simulink model "fixed_point_model"  (R2022b)
settings: Solver=FixedStepDiscrete  StartTime=0.0  StopTime=0.01  FixedStep=1e-10  RelTol=1e-3
undefined symbols (not defined in the file or in its folder): theta_input
libraries: dspsigops x206, dspsrcs4 x16, simulink x8, commdigbbndpm3 x1, commrandsrc3 x1
(part 1 of 6)
settings Model: FPTShortcutValueString='{{},{''BaselineRun'',1,1,1,''BaselineRun'','''',{},''M'','''',''''}}'  Creator=ASAA  LastModifiedBy=ASAA
settings DataIOCC: SaveOutput=off  SignalLogging=off  DSMLogging=off  ReturnWorkspaceOutputs=off
settings DebuggingCC: SignalRangeChecking=warning  UnderSpecifiedDimensionMsg=warning

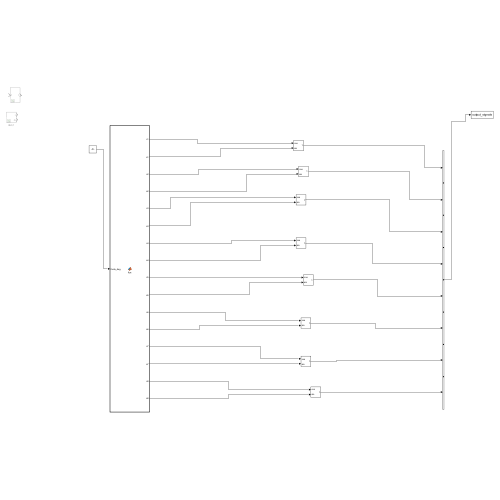
[thumbnail: Simulink's stored preview of the top-level diagram]
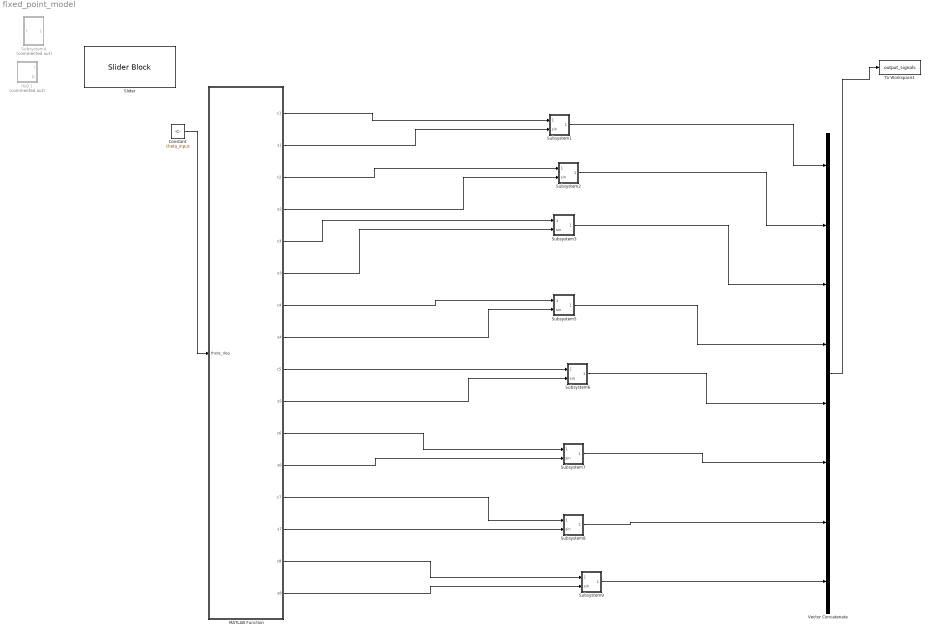
== system fixed_point_model ==
  Constant : Constant  Value=theta_input
  I&Q 1 : Subsystem  Commented=on
  MATLAB Function : MATLAB Function  TreatAsAtomicUnit=on
  Slider : SliderBlock
  Subsystem1 : Subsystem
  Subsystem2 : Subsystem
  Subsystem3 : Subsystem
  Subsystem4 : Subsystem  Commented=on
  Subsystem5 : Subsystem
  Subsystem6 : Subsystem
  Subsystem7 : Subsystem
  Subsystem8 : Subsystem
  Subsystem9 : Subsystem
  To Workspace1 : ToWorkspace  VariableName=output_signals  SampleTime=-1
  Vector Concatenate : Concatenate  NumInputs=8
  wires:
  Constant/1 -> MATLAB Function/1(theta_deg)
  Vector Concatenate/1 -> To Workspace1/1
  MATLAB Function/1(c1) -> Subsystem1/1(cos)
  MATLAB Function/2(s1) -> Subsystem1/2(sin)
  Subsystem1/1(Out1) -> Vector Concatenate/1
  MATLAB Function/3(c2) -> Subsystem2/1(cos)
  MATLAB Function/4(s2) -> Subsystem2/2(sin)
  MATLAB Function/5(c3) -> Subsystem3/1(cos)
  MATLAB Function/6(s3) -> Subsystem3/2(sin)
  MATLAB Function/7(c4) -> Subsystem5/1(cos)
  MATLAB Function/8(s4) -> Subsystem5/2(sin)
  Subsystem5/1(Out1) -> Vector Concatenate/4
  MATLAB Function/9(c5) -> Subsystem6/1(cos)
  MATLAB Function/10(s5) -> Subsystem6/2(sin)
  Subsystem6/1(Out1) -> Vector Concatenate/5
  MATLAB Function/13(c7) -> Subsystem8/1(cos)
  MATLAB Function/14(s7) -> Subsystem8/2(sin)
  Subsystem8/1(Out1) -> Vector Concatenate/7
  MATLAB Function/16(s8) -> Subsystem9/2(sin)
  MATLAB Function/15(c8) -> Subsystem9/1(cos)
  Subsystem9/1(Out1) -> Vector Concatenate/8
  Subsystem2/1(Out1) -> Vector Concatenate/2
  Subsystem3/1(Out1) -> Vector Concatenate/3
  Subsystem7/1(Out1) -> Vector Concatenate/6
  MATLAB Function/11(c6) -> Subsystem7/1(cos)
  MATLAB Function/12(s6) -> Subsystem7/2(sin)

== system fixed_point_model/I&Q 1 ==
  Complex to Real-Imag : ComplexToRealImag
  QPSK Modulator Baseband : commdigbbndpm3/QPSK Modulator Baseband  InType=Integer  Enc=Gray  Ph=pi/2  outDtype=double  outWordLen=16  outUDDataType=sfix(16)  outFracLenMode=Best precision  outFracLen=15  outDataTypeStr=double  outLastDataTypeStr=double
  Random Integer Generator : commrandsrc3/Random Integer Generator  SetSize=4  SeedSource=Auto  Seed=0  SampleTime=1/3.125e6  SamplesPerFrame=1  OutputDataType=double  SimulateUsing=Interpreted execution
  I : Outport
  Q : Outport  Port=2
  wires:
  QPSK Modulator Baseband/1 -> Complex to Real-Imag/1
  Random Integer Generator/1 -> QPSK Modulator Baseband/1
  Complex to Real-Imag/1 -> I/1
  Complex to Real-Imag/2 -> Q/1

== system fixed_point_model/Subsystem1 ==
  cos : Inport
  sin : Inport  Port=2
  Real-Imag to Complex : RealImagToComplex  Commented=on
  Sine Wave : Subsystem  Tag=DecoupledSystem
  Sine Wave1 : Subsystem  Tag=DecoupledSystem
  Subsystem : Subsystem
  Subsystem1 : Subsystem
  Subsystem2 : Subsystem
  Subsystem3 : Subsystem
  filter_with_comb1 : Subsystem
  filter_with_comb2 : Subsystem
  Out1 : Outport
      settings: SignalType=complex
  wires:
  filter_with_comb1/1(I') -> Subsystem2/1(In1)
  filter_with_comb2/1(I') -> Subsystem3/1(In1)
  Subsystem3/1(Q) -> Subsystem/1(Q), Real-Imag to Complex/2
  Subsystem2/1(Q) -> Subsystem/2(In2), Real-Imag to Complex/1
  Sine Wave/1(I) -> Subsystem1/1(I)
  Sine Wave1/1(Q) -> Subsystem1/2(Q)
  Subsystem1/1(Q') -> filter_with_comb2/1(Q'1)
  Subsystem1/2(I') -> filter_with_comb1/1(Q'1)
  sin/1 -> Subsystem1/4(sin)
  cos/1 -> Subsystem1/3(cos)
  Subsystem/1(Out1) -> Out1/1

== system fixed_point_model/Subsystem2 ==
  cos : Inport
  sin : Inport  Port=2
  Real-Imag to Complex : RealImagToComplex  Commented=on
  Sine Wave : Subsystem  Tag=DecoupledSystem
  Sine Wave1 : Subsystem  Tag=DecoupledSystem
  Subsystem : Subsystem
  Subsystem1 : Subsystem
  Subsystem2 : Subsystem
  Subsystem3 : Subsystem
  filter_with_comb1 : Subsystem
  filter_with_comb2 : Subsystem
  Out1 : Outport
      settings: SignalType=complex
  wires:
  filter_with_comb1/1(I') -> Subsystem2/1(In1)
  filter_with_comb2/1(I') -> Subsystem3/1(In1)
  Subsystem3/1(Q) -> Subsystem/1(Q), Real-Imag to Complex/2
  Subsystem2/1(Q) -> Subsystem/2(In2), Real-Imag to Complex/1
  Sine Wave/1(I) -> Subsystem1/1(I)
  Sine Wave1/1(Q) -> Subsystem1/2(Q)
  Subsystem1/1(Q') -> filter_with_comb2/1(Q'1)
  Subsystem1/2(I') -> filter_with_comb1/1(Q'1)
  sin/1 -> Subsystem1/4(sin)
  cos/1 -> Subsystem1/3(cos)
  Subsystem/1(Out1) -> Out1/1

== system fixed_point_model/Subsystem3 ==
  cos : Inport
  sin : Inport  Port=2
  Real-Imag to Complex : RealImagToComplex  Commented=on
  Sine Wave : Subsystem  Tag=DecoupledSystem
  Sine Wave1 : Subsystem  Tag=DecoupledSystem
  Subsystem : Subsystem
  Subsystem1 : Subsystem
  Subsystem2 : Subsystem
  Subsystem3 : Subsystem
  filter_with_comb1 : Subsystem
  filter_with_comb2 : Subsystem
  Out1 : Outport
      settings: SignalType=complex
  wires:
  filter_with_comb1/1(I') -> Subsystem2/1(In1)
  filter_with_comb2/1(I') -> Subsystem3/1(In1)
  Subsystem3/1(Q) -> Subsystem/1(Q), Real-Imag to Complex/2
  Subsystem2/1(Q) -> Subsystem/2(In2), Real-Imag to Complex/1
  Sine Wave/1(I) -> Subsystem1/1(I)
  Sine Wave1/1(Q) -> Subsystem1/2(Q)
  Subsystem1/1(Q') -> filter_with_comb2/1(Q'1)
  Subsystem1/2(I') -> filter_with_comb1/1(Q'1)
  sin/1 -> Subsystem1/4(sin)
  cos/1 -> Subsystem1/3(cos)
  Subsystem/1(Out1) -> Out1/1

== system fixed_point_model/Subsystem4 ==
  I' : Inport
  stage2 : Subsystem
  stage_1 : Subsystem
  stage_2 : Subsystem
  stage_3 : Subsystem
  stage_4 : Subsystem
  stage_5 : Subsystem
  Out1 : Outport
  wires:
  stage_2/1(Out1) -> stage_4/1(In1)
  I'/1 -> stage_1/1(In1)
  stage_1/1(Out1) -> stage_2/1(In1)
  stage_4/1(Out1) -> Out1/1

== system fixed_point_model/Subsystem5 ==
  cos : Inport
  sin : Inport  Port=2
  Real-Imag to Complex : RealImagToComplex  Commented=on
  Sine Wave : Subsystem  Tag=DecoupledSystem
  Sine Wave1 : Subsystem  Tag=DecoupledSystem
  Subsystem : Subsystem
  Subsystem1 : Subsystem
  Subsystem2 : Subsystem
  Subsystem3 : Subsystem
  filter_with_comb1 : Subsystem
  filter_with_comb2 : Subsystem
  Out1 : Outport
      settings: SignalType=complex
  wires:
  filter_with_comb1/1(I') -> Subsystem2/1(In1)
  filter_with_comb2/1(I') -> Subsystem3/1(In1)
  Subsystem3/1(Q) -> Subsystem/1(Q), Real-Imag to Complex/2
  Subsystem2/1(Q) -> Subsystem/2(In2), Real-Imag to Complex/1
  Sine Wave/1(I) -> Subsystem1/1(I)
  Sine Wave1/1(Q) -> Subsystem1/2(Q)
  Subsystem1/1(Q') -> filter_with_comb2/1(Q'1)
  Subsystem1/2(I') -> filter_with_comb1/1(Q'1)
  sin/1 -> Subsystem1/4(sin)
  cos/1 -> Subsystem1/3(cos)
  Subsystem/1(Out1) -> Out1/1

== system fixed_point_model/Subsystem6 ==
  cos : Inport
  sin : Inport  Port=2
  Real-Imag to Complex : RealImagToComplex  Commented=on
  Sine Wave : Subsystem  Tag=DecoupledSystem
  Sine Wave1 : Subsystem  Tag=DecoupledSystem
  Subsystem : Subsystem
  Subsystem1 : Subsystem
  Subsystem2 : Subsystem
  Subsystem3 : Subsystem
  filter_with_comb1 : Subsystem
  filter_with_comb2 : Subsystem
  Out1 : Outport
      settings: SignalType=complex
  wires:
  filter_with_comb1/1(I') -> Subsystem2/1(In1)
  filter_with_comb2/1(I') -> Subsystem3/1(In1)
  Subsystem3/1(Q) -> Subsystem/1(Q), Real-Imag to Complex/2
  Subsystem2/1(Q) -> Subsystem/2(In2), Real-Imag to Complex/1
  Sine Wave/1(I) -> Subsystem1/1(I)
  Sine Wave1/1(Q) -> Subsystem1/2(Q)
  Subsystem1/1(Q') -> filter_with_comb2/1(Q'1)
  Subsystem1/2(I') -> filter_with_comb1/1(Q'1)
  sin/1 -> Subsystem1/4(sin)
  cos/1 -> Subsystem1/3(cos)
  Subsystem/1(Out1) -> Out1/1

== system fixed_point_model/Subsystem7 ==
  cos : Inport
  sin : Inport  Port=2
  Real-Imag to Complex : RealImagToComplex  Commented=on
  Sine Wave : Subsystem  Tag=DecoupledSystem
  Sine Wave1 : Subsystem  Tag=DecoupledSystem
  Subsystem : Subsystem
  Subsystem1 : Subsystem
  Subsystem2 : Subsystem
  Subsystem3 : Subsystem
  filter_with_comb1 : Subsystem
  filter_with_comb2 : Subsystem
  Out1 : Outport
      settings: SignalType=complex
  wires:
  filter_with_comb1/1(I') -> Subsystem2/1(In1)
  filter_with_comb2/1(I') -> Subsystem3/1(In1)
  Subsystem3/1(Q) -> Subsystem/1(Q), Real-Imag to Complex/2
  Subsystem2/1(Q) -> Subsystem/2(In2), Real-Imag to Complex/1
  Sine Wave/1(I) -> Subsystem1/1(I)
  Sine Wave1/1(Q) -> Subsystem1/2(Q)
  Subsystem1/1(Q') -> filter_with_comb2/1(Q'1)
  Subsystem1/2(I') -> filter_with_comb1/1(Q'1)
  sin/1 -> Subsystem1/4(sin)
  cos/1 -> Subsystem1/3(cos)
  Subsystem/1(Out1) -> Out1/1

== system fixed_point_model/Subsystem8 ==
  cos : Inport
  sin : Inport  Port=2
  Real-Imag to Complex : RealImagToComplex  Commented=on
  Sine Wave : Subsystem  Tag=DecoupledSystem
  Sine Wave1 : Subsystem  Tag=DecoupledSystem
  Subsystem : Subsystem
  Subsystem1 : Subsystem
  Subsystem2 : Subsystem
  Subsystem3 : Subsystem
  filter_with_comb1 : Subsystem
  filter_with_comb2 : Subsystem
  Out1 : Outport
      settings: SignalType=complex
  wires:
  filter_with_comb1/1(I') -> Subsystem2/1(In1)
  filter_with_comb2/1(I') -> Subsystem3/1(In1)
  Subsystem3/1(Q) -> Subsystem/1(Q), Real-Imag to Complex/2
  Subsystem2/1(Q) -> Subsystem/2(In2), Real-Imag to Complex/1
  Sine Wave/1(I) -> Subsystem1/1(I)
  Sine Wave1/1(Q) -> Subsystem1/2(Q)
  Subsystem1/1(Q') -> filter_with_comb2/1(Q'1)
  Subsystem1/2(I') -> filter_with_comb1/1(Q'1)
  sin/1 -> Subsystem1/4(sin)
  cos/1 -> Subsystem1/3(cos)
  Subsystem/1(Out1) -> Out1/1

== system fixed_point_model/Subsystem9 ==
  cos : Inport
  sin : Inport  Port=2
  Real-Imag to Complex : RealImagToComplex  Commented=on
  Sine Wave : Subsystem  Tag=DecoupledSystem
  Sine Wave1 : Subsystem  Tag=DecoupledSystem
  Subsystem : Subsystem
  Subsystem1 : Subsystem
  Subsystem2 : Subsystem
  Subsystem3 : Subsystem
  filter_with_comb1 : Subsystem
  filter_with_comb2 : Subsystem
  Out1 : Outport
      settings: SignalType=complex
  wires:
  filter_with_comb1/1(I') -> Subsystem2/1(In1)
  filter_with_comb2/1(I') -> Subsystem3/1(In1)
  Subsystem3/1(Q) -> Subsystem/1(Q), Real-Imag to Complex/2
  Subsystem2/1(Q) -> Subsystem/2(In2), Real-Imag to Complex/1
  Sine Wave/1(I) -> Subsystem1/1(I)
  Sine Wave1/1(Q) -> Subsystem1/2(Q)
  Subsystem1/1(Q') -> filter_with_comb2/1(Q'1)
  Subsystem1/2(I') -> filter_with_comb1/1(Q'1)
  sin/1 -> Subsystem1/4(sin)
  cos/1 -> Subsystem1/3(cos)
  Subsystem/1(Out1) -> Out1/1

== system fixed_point_model/Subsystem1/Sine Wave ==
  ReplicaOfSource : dspsrcs4/Sine Wave  Amplitude=0.631  Frequency=100e3  Phase=0  SampleMode=Discrete  OutComplex=Real  CompMethod=Trigonometric fcn  TableSize=Speed  SampleTime=1/3.125e6  SamplesPerFrame=1  ResetState=Restart at time zero  OutputFrames=off  dataType=double  wordLen=16  udDataType=sfix(16)  fracBitsMode=Best precision  numFracBits=15  OutDataTypeStr=double  LastOutDataTypeStr=double
  I : Outport  LockScale=on
  wires:
  ReplicaOfSource/1 -> I/1

== system fixed_point_model/Subsystem1/Sine Wave1 ==
  ReplicaOfSource : dspsrcs4/Sine Wave  Amplitude=0.631  Frequency=100e3  Phase=pi/2  SampleMode=Discrete  OutComplex=Real  CompMethod=Trigonometric fcn  TableSize=Speed  SampleTime=1/3.125e6  SamplesPerFrame=1  ResetState=Restart at time zero  OutputFrames=off  dataType=double  wordLen=16  udDataType=sfix(16)  fracBitsMode=Best precision  numFracBits=15  OutDataTypeStr=double  LastOutDataTypeStr=double
  Q : Outport  LockScale=on
  wires:
  ReplicaOfSource/1 -> Q/1

== system fixed_point_model/Subsystem1/Subsystem ==
  Q : Inport
  In2 : Inport  Port=2
  -I(t) : Gain  Gain=-1
  -Q(t) : Gain  Gain=-1
  Counter : simulink/Sources/Counter Limited  uplimit=3  tsamp=1/400e6
  Multiport Switch (MUX) : MultiPortSwitch  DataPortOrder=Zero-based contiguous  Inputs=4  zeroidx=on  SaturateOnIntegerOverflow=off  InputSameDT=off
  Out1 : Outport
  wires:
  Q/1 -> Multiport Switch (MUX)/2, -I(t)/1
  Counter/1 -> Multiport Switch (MUX)/1
  -Q(t)/1 -> Multiport Switch (MUX)/3
  In2/1 -> Multiport Switch (MUX)/5, -Q(t)/1
  -I(t)/1 -> Multiport Switch (MUX)/4
  Multiport Switch (MUX)/1 -> Out1/1

== system fixed_point_model/Subsystem1/Subsystem1 ==
  I : Inport
  Q : Inport  Port=2
  cos : Inport  Port=3
  sin : Inport  Port=4
  Add : Sum  Inputs=+-
  Product{,1..3} (4 alike) : Product
  Subtract : Sum
  Q' : Outport
  I' : Outport  Port=2
  wires:
  sin/1 -> Product/2, Product1/2
  Add/1 -> Q'/1
  Product3/1 -> Add/1
  Product2/1 -> Subtract/1
  Product1/1 -> Add/2
  Product/1 -> Subtract/2
  Subtract/1 -> I'/1
  I/1 -> Product1/1, Product2/2
  Q/1 -> Product3/2, Product/1
  cos/1 -> Product2/1, Product3/1

== system fixed_point_model/Subsystem1/Subsystem2 ==
  In1 : Inport
  Gain : Gain  Gain=2  SaturateOnIntegerOverflow=on
  Sign : Signum
  Sum : Sum  Inputs=|+-  RndMeth=Nearest  SaturateOnIntegerOverflow=on
  Sum1 : Sum  Inputs=|++-  SaturateOnIntegerOverflow=on
  Unit Delay : UnitDelay  InputProcessing=Columns as channels (frame based)  SampleTime=1e-8  HasFrameUpgradeWarning=on
  Unit Delay1 : UnitDelay  InputProcessing=Columns as channels (frame based)  SampleTime=1e-8  HasFrameUpgradeWarning=on
  Q : Outport
  wires:
  Sign/1 -> Q/1, Sum/2
  Sum1/1 -> Sign/1, Sum/1
  Sum/1 -> Unit Delay1/1
  Unit Delay1/1 -> Unit Delay/1, Gain/1
  Gain/1 -> Sum1/2
  In1/1 -> Sum1/1
  Unit Delay/1 -> Sum1/3

== system fixed_point_model/Subsystem1/Subsystem3 ==
  In1 : Inport
  Gain : Gain  Gain=2  SaturateOnIntegerOverflow=on
  Sign : Signum
  Sum : Sum  Inputs=|+-  RndMeth=Nearest  SaturateOnIntegerOverflow=on
  Sum1 : Sum  Inputs=|++-  SaturateOnIntegerOverflow=on
  Unit Delay : UnitDelay  InputProcessing=Columns as channels (frame based)  SampleTime=1e-8  HasFrameUpgradeWarning=on
  Unit Delay1 : UnitDelay  InputProcessing=Columns as channels (frame based)  SampleTime=1e-8  HasFrameUpgradeWarning=on
  Q : Outport
  wires:
  Sign/1 -> Q/1, Sum/2
  Sum1/1 -> Sign/1, Sum/1
  Sum/1 -> Unit Delay1/1
  Unit Delay1/1 -> Unit Delay/1, Gain/1
  Gain/1 -> Sum1/2
  In1/1 -> Sum1/1
  Unit Delay/1 -> Sum1/3

== system fixed_point_model/Subsystem1/filter_with_comb1 ==
  Q'1 : Inport
  Gain : Gain  Gain=1/512
  Stage_1 : Subsystem
  stage_3 : Subsystem
  stage_4 : Subsystem
  I' : Outport
  wires:
  stage_4/1(Out1) -> stage_3/1(In1)
  stage_3/1(Q') -> Stage_1/1(In1)
  Stage_1/1(Out1) -> Gain/1
  Gain/1 -> I'/1
  Q'1/1 -> stage_4/1(Q')

== system fixed_point_model/Subsystem1/filter_with_comb2 ==
  Q'1 : Inport
  Gain : Gain  Gain=1/512
  Stage_1 : Subsystem
  stage_3 : Subsystem
  stage_4 : Subsystem
  I' : Outport
  wires:
  stage_4/1(Out1) -> stage_3/1(In1)
  stage_3/1(Q') -> Stage_1/1(In1)
  Stage_1/1(Out1) -> Gain/1
  Gain/1 -> I'/1
  Q'1/1 -> stage_4/1(Q')

== system fixed_point_model/Subsystem2/Sine Wave ==
  ReplicaOfSource : dspsrcs4/Sine Wave  Amplitude=0.631  Frequency=100e3  Phase=0  SampleMode=Discrete  OutComplex=Real  CompMethod=Trigonometric fcn  TableSize=Speed  SampleTime=1/3.125e6  SamplesPerFrame=1  ResetState=Restart at time zero  OutputFrames=off  dataType=double  wordLen=16  udDataType=sfix(16)  fracBitsMode=Best precision  numFracBits=15  OutDataTypeStr=double  LastOutDataTypeStr=double
  I : Outport  LockScale=on
  wires:
  ReplicaOfSource/1 -> I/1

== system fixed_point_model/Subsystem2/Sine Wave1 ==
  ReplicaOfSource : dspsrcs4/Sine Wave  Amplitude=0.631  Frequency=100e3  Phase=pi/2  SampleMode=Discrete  OutComplex=Real  CompMethod=Trigonometric fcn  TableSize=Speed  SampleTime=1/3.125e6  SamplesPerFrame=1  ResetState=Restart at time zero  OutputFrames=off  dataType=double  wordLen=16  udDataType=sfix(16)  fracBitsMode=Best precision  numFracBits=15  OutDataTypeStr=double  LastOutDataTypeStr=double
  Q : Outport  LockScale=on
  wires:
  ReplicaOfSource/1 -> Q/1

== system fixed_point_model/Subsystem2/Subsystem ==
  Q : Inport
  In2 : Inport  Port=2
  -I(t) : Gain  Gain=-1
  -Q(t) : Gain  Gain=-1
  Counter : simulink/Sources/Counter Limited  uplimit=3  tsamp=1/400e6
  Multiport Switch (MUX) : MultiPortSwitch  DataPortOrder=Zero-based contiguous  Inputs=4  zeroidx=on  SaturateOnIntegerOverflow=off  InputSameDT=off
  Out1 : Outport
  wires:
  Q/1 -> Multiport Switch (MUX)/2, -I(t)/1
  Counter/1 -> Multiport Switch (MUX)/1
  -Q(t)/1 -> Multiport Switch (MUX)/3
  In2/1 -> Multiport Switch (MUX)/5, -Q(t)/1
  -I(t)/1 -> Multiport Switch (MUX)/4
  Multiport Switch (MUX)/1 -> Out1/1

== system fixed_point_model/Subsystem2/Subsystem1 ==
  I : Inport
  Q : Inport  Port=2
  cos : Inport  Port=3
  sin : Inport  Port=4
  Add : Sum  Inputs=+-
  Product{,1..3} (4 alike) : Product
  Subtract : Sum
  Q' : Outport
  I' : Outport  Port=2
  wires:
  sin/1 -> Product/2, Product1/2
  Add/1 -> Q'/1
  Product3/1 -> Add/1
  Product2/1 -> Subtract/1
  Product1/1 -> Add/2
  Product/1 -> Subtract/2
  Subtract/1 -> I'/1
  I/1 -> Product1/1, Product2/2
  Q/1 -> Product3/2, Product/1
  cos/1 -> Product2/1, Product3/1

== system fixed_point_model/Subsystem2/Subsystem2 ==
  In1 : Inport
  Gain : Gain  Gain=2  SaturateOnIntegerOverflow=on
  Sign : Signum
  Sum : Sum  Inputs=|+-  RndMeth=Nearest  SaturateOnIntegerOverflow=on
  Sum1 : Sum  Inputs=|++-  SaturateOnIntegerOverflow=on
  Unit Delay : UnitDelay  InputProcessing=Columns as channels (frame based)  SampleTime=1e-8  HasFrameUpgradeWarning=on
  Unit Delay1 : UnitDelay  InputProcessing=Columns as channels (frame based)  SampleTime=1e-8  HasFrameUpgradeWarning=on
  Q : Outport
  wires:
  Sign/1 -> Q/1, Sum/2
  Sum1/1 -> Sign/1, Sum/1
  Sum/1 -> Unit Delay1/1
  Unit Delay1/1 -> Unit Delay/1, Gain/1
  Gain/1 -> Sum1/2
  In1/1 -> Sum1/1
  Unit Delay/1 -> Sum1/3

== system fixed_point_model/Subsystem2/Subsystem3 ==
  In1 : Inport
  Gain : Gain  Gain=2  SaturateOnIntegerOverflow=on
  Sign : Signum
  Sum : Sum  Inputs=|+-  RndMeth=Nearest  SaturateOnIntegerOverflow=on
  Sum1 : Sum  Inputs=|++-  SaturateOnIntegerOverflow=on
  Unit Delay : UnitDelay  InputProcessing=Columns as channels (frame based)  SampleTime=1e-8  HasFrameUpgradeWarning=on
  Unit Delay1 : UnitDelay  InputProcessing=Columns as channels (frame based)  SampleTime=1e-8  HasFrameUpgradeWarning=on
  Q : Outport
  wires:
  Sign/1 -> Q/1, Sum/2
  Sum1/1 -> Sign/1, Sum/1
  Sum/1 -> Unit Delay1/1
  Unit Delay1/1 -> Unit Delay/1, Gain/1
  Gain/1 -> Sum1/2
  In1/1 -> Sum1/1
  Unit Delay/1 -> Sum1/3

== system fixed_point_model/Subsystem2/filter_with_comb1 ==
  Q'1 : Inport
  Gain : Gain  Gain=1/512
  Stage_1 : Subsystem
  stage_3 : Subsystem
  stage_4 : Subsystem
  I' : Outport
  wires:
  stage_4/1(Out1) -> stage_3/1(In1)
  stage_3/1(Q') -> Stage_1/1(In1)
  Stage_1/1(Out1) -> Gain/1
  Gain/1 -> I'/1
  Q'1/1 -> stage_4/1(Q')

== system fixed_point_model/Subsystem2/filter_with_comb2 ==
  Q'1 : Inport
  Gain : Gain  Gain=1/512
  Stage_1 : Subsystem
  stage_3 : Subsystem
  stage_4 : Subsystem
  I' : Outport
  wires:
  stage_4/1(Out1) -> stage_3/1(In1)
  stage_3/1(Q') -> Stage_1/1(In1)
  Stage_1/1(Out1) -> Gain/1
  Gain/1 -> I'/1
  Q'1/1 -> stage_4/1(Q')

== system fixed_point_model/Subsystem3/Sine Wave ==
  ReplicaOfSource : dspsrcs4/Sine Wave  Amplitude=0.631  Frequency=100e3  Phase=0  SampleMode=Discrete  OutComplex=Real  CompMethod=Trigonometric fcn  TableSize=Speed  SampleTime=1/3.125e6  SamplesPerFrame=1  ResetState=Restart at time zero  OutputFrames=off  dataType=double  wordLen=16  udDataType=sfix(16)  fracBitsMode=Best precision  numFracBits=15  OutDataTypeStr=double  LastOutDataTypeStr=double
  I : Outport  LockScale=on
  wires:
  ReplicaOfSource/1 -> I/1

== system fixed_point_model/Subsystem3/Sine Wave1 ==
  ReplicaOfSource : dspsrcs4/Sine Wave  Amplitude=0.631  Frequency=100e3  Phase=pi/2  SampleMode=Discrete  OutComplex=Real  CompMethod=Trigonometric fcn  TableSize=Speed  SampleTime=1/3.125e6  SamplesPerFrame=1  ResetState=Restart at time zero  OutputFrames=off  dataType=double  wordLen=16  udDataType=sfix(16)  fracBitsMode=Best precision  numFracBits=15  OutDataTypeStr=double  LastOutDataTypeStr=double
  Q : Outport  LockScale=on
  wires:
  ReplicaOfSource/1 -> Q/1

== system fixed_point_model/Subsystem3/Subsystem ==
  Q : Inport
  In2 : Inport  Port=2
  -I(t) : Gain  Gain=-1
  -Q(t) : Gain  Gain=-1
  Counter : simulink/Sources/Counter Limited  uplimit=3  tsamp=1/400e6
  Multiport Switch (MUX) : MultiPortSwitch  DataPortOrder=Zero-based contiguous  Inputs=4  zeroidx=on  SaturateOnIntegerOverflow=off  InputSameDT=off
  Out1 : Outport
  wires:
  Q/1 -> Multiport Switch (MUX)/2, -I(t)/1
  Counter/1 -> Multiport Switch (MUX)/1
  -Q(t)/1 -> Multiport Switch (MUX)/3
  In2/1 -> Multiport Switch (MUX)/5, -Q(t)/1
  -I(t)/1 -> Multiport Switch (MUX)/4
  Multiport Switch (MUX)/1 -> Out1/1

== system fixed_point_model/Subsystem3/Subsystem1 ==
  I : Inport
  Q : Inport  Port=2
  cos : Inport  Port=3
  sin : Inport  Port=4
  Add : Sum  Inputs=+-
  Product{,1..3} (4 alike) : Product
  Subtract : Sum
  Q' : Outport
  I' : Outport  Port=2
  wires:
  sin/1 -> Product/2, Product1/2
  Add/1 -> Q'/1
  Product3/1 -> Add/1
  Product2/1 -> Subtract/1
  Product1/1 -> Add/2
  Product/1 -> Subtract/2
  Subtract/1 -> I'/1
  I/1 -> Product1/1, Product2/2
  Q/1 -> Product3/2, Product/1
  cos/1 -> Product2/1, Product3/1

== system fixed_point_model/Subsystem3/Subsystem2 ==
  In1 : Inport
  Gain : Gain  Gain=2  SaturateOnIntegerOverflow=on
  Sign : Signum
  Sum : Sum  Inputs=|+-  RndMeth=Nearest  SaturateOnIntegerOverflow=on
  Sum1 : Sum  Inputs=|++-  SaturateOnIntegerOverflow=on
  Unit Delay : UnitDelay  InputProcessing=Columns as channels (frame based)  SampleTime=1e-8  HasFrameUpgradeWarning=on
  Unit Delay1 : UnitDelay  InputProcessing=Columns as channels (frame based)  SampleTime=1e-8  HasFrameUpgradeWarning=on
  Q : Outport
  wires:
  Sign/1 -> Q/1, Sum/2
  Sum1/1 -> Sign/1, Sum/1
  Sum/1 -> Unit Delay1/1
  Unit Delay1/1 -> Unit Delay/1, Gain/1
  Gain/1 -> Sum1/2
  In1/1 -> Sum1/1
  Unit Delay/1 -> Sum1/3

== system fixed_point_model/Subsystem3/Subsystem3 ==
  In1 : Inport
  Gain : Gain  Gain=2  SaturateOnIntegerOverflow=on
  Sign : Signum
  Sum : Sum  Inputs=|+-  RndMeth=Nearest  SaturateOnIntegerOverflow=on
  Sum1 : Sum  Inputs=|++-  SaturateOnIntegerOverflow=on
  Unit Delay : UnitDelay  InputProcessing=Columns as channels (frame based)  SampleTime=1e-8  HasFrameUpgradeWarning=on
  Unit Delay1 : UnitDelay  InputProcessing=Columns as channels (frame based)  SampleTime=1e-8  HasFrameUpgradeWarning=on
  Q : Outport
  wires:
  Sign/1 -> Q/1, Sum/2
  Sum1/1 -> Sign/1, Sum/1
  Sum/1 -> Unit Delay1/1
  Unit Delay1/1 -> Unit Delay/1, Gain/1
  Gain/1 -> Sum1/2
  In1/1 -> Sum1/1
  Unit Delay/1 -> Sum1/3

== system fixed_point_model/Subsystem3/filter_with_comb1 ==
  Q'1 : Inport
  Gain : Gain  Gain=1/512
  Stage_1 : Subsystem
  stage_3 : Subsystem
  stage_4 : Subsystem
  I' : Outport
  wires:
  stage_4/1(Out1) -> stage_3/1(In1)
  stage_3/1(Q') -> Stage_1/1(In1)
  Stage_1/1(Out1) -> Gain/1
  Gain/1 -> I'/1
  Q'1/1 -> stage_4/1(Q')

== system fixed_point_model/Subsystem3/filter_with_comb2 ==
  Q'1 : Inport
  Gain : Gain  Gain=1/512
  Stage_1 : Subsystem
  stage_3 : Subsystem
  stage_4 : Subsystem
  I' : Outport
  wires:
  stage_4/1(Out1) -> stage_3/1(In1)
  stage_3/1(Q') -> Stage_1/1(In1)
  Stage_1/1(Out1) -> Gain/1
  Gain/1 -> I'/1
  Q'1/1 -> stage_4/1(Q')

== system fixed_point_model/Subsystem4/stage2 ==
  In1 : Inport
  Add : Sum  Inputs=++++
  Delay2 : Delay  InitialCondition=0
  Delay3 : Delay  DelayLength=3  InitialCondition=0
  Delay4 : Delay  DelayLength=1  InitialCondition=0
  Subsystem : Subsystem
  Subsystem1 : Subsystem
  Subsystem2 : Subsystem
  Subsystem3 : Subsystem
  Upsample{,1..3} (4 alike) : dspsigops/Upsample  N=4  phase=0  InputProcessing=Columns as channels (frame based)  RateOptions=Enforce single-rate processing  ic=0  mode=Unused parameter value
  Out1 : Outport
  wires:
  In1/1 -> Subsystem3/1(In1), Subsystem2/1(In1), Subsystem1/1(In1), Subsystem/1(In1)
  Add/1 -> Out1/1
  Upsample2/1 -> Delay3/1
  Upsample3/1 -> Add/4
  Upsample/1 -> Delay4/1
  Upsample1/1 -> Delay2/1
  Subsystem3/1(Out1) -> Upsample2/1
  Subsystem2/1(Out1) -> Upsample1/1
  Subsystem1/1(Out1) -> Upsample/1
  Subsystem/1(Out1) -> Upsample3/1
  Delay4/1 -> Add/1
  Delay2/1 -> Add/2
  Delay3/1 -> Add/3

== system fixed_point_model/Subsystem4/stage_1 ==
  In1 : Inport
  Add : Sum
  Delay1 : Delay  DelayLength=7  InitialCondition=0
  Delay2 : Delay  DelayLength=1  InitialCondition=0
  Gain : Gain  Gain=0.5000
  Subsystem1 : Subsystem
  Upsample : dspsigops/Upsample  N=2  phase=0  InputProcessing=Columns as channels (frame based)  RateOptions=Enforce single-rate processing  ic=0  mode=Unused parameter value
  Upsample1 : dspsigops/Upsample  N=2  phase=0  InputProcessing=Columns as channels (frame based)  RateOptions=Enforce single-rate processing  ic=0  mode=Unused parameter value
  Out1 : Outport
  wires:
  Add/1 -> Out1/1
  Delay2/1 -> Add/2
  Upsample1/1 -> Delay2/1
  In1/1 -> Delay1/1, Subsystem1/1(In1)
  Delay1/1 -> Gain/1
  Subsystem1/1(Out2) -> Upsample/1
  Upsample/1 -> Add/1
  Gain/1 -> Upsample1/1

== system fixed_point_model/Subsystem4/stage_2 ==
  In1 : Inport
  Add1 : Sum
  Delay3 : Delay  DelayLength=4  InitialCondition=0
  Delay4 : Delay  DelayLength=1  InitialCondition=0
  Gain1 : Gain  Gain=0.5000
  Subsystem : Subsystem
  Upsample2 : dspsigops/Upsample  N=2  phase=0  InputProcessing=Columns as channels (frame based)  RateOptions=Enforce single-rate processing  ic=0  mode=Unused parameter value
  Upsample3 : dspsigops/Upsample  N=2  phase=0  InputProcessing=Columns as channels (frame based)  RateOptions=Enforce single-rate processing  ic=0  mode=Unused parameter value
  Out1 : Outport
  wires:
  Upsample2/1 -> Delay4/1
  In1/1 -> Subsystem/1(In1), Delay3/1
  Gain1/1 -> Upsample2/1
  Add1/1 -> Out1/1
  Delay3/1 -> Gain1/1
  Upsample3/1 -> Add1/1
  Delay4/1 -> Add1/2
  Subsystem/1(Out1) -> Upsample3/1

== system fixed_point_model/Subsystem4/stage_3 ==
  In1 : Inport
  Add1 : Sum
  Delay3 : Delay  DelayLength=4  InitialCondition=0
  Delay4 : Delay  DelayLength=1  InitialCondition=0
  Gain1 : Gain  Gain=0.5000
  Subsystem : Subsystem
  Upsample2 : dspsigops/Upsample  N=2  phase=0  InputProcessing=Columns as channels (frame based)  RateOptions=Enforce single-rate processing  ic=0  mode=Unused parameter value
  Upsample3 : dspsigops/Upsample  N=2  phase=0  InputProcessing=Columns as channels (frame based)  RateOptions=Enforce single-rate processing  ic=0  mode=Unused parameter value
  Out1 : Outport
  wires:
  Upsample2/1 -> Delay4/1
  In1/1 -> Subsystem/1(In1), Delay3/1
  Gain1/1 -> Upsample2/1
  Add1/1 -> Out1/1
  Delay3/1 -> Gain1/1
  Upsample3/1 -> Add1/1
  Delay4/1 -> Add1/2
  Subsystem/1(Out1) -> Upsample3/1

== system fixed_point_model/Subsystem4/stage_4 ==
  In1 : Inport
  Add1 : Sum
  Delay3 : Delay  DelayLength=4  InitialCondition=0
  Delay4 : Delay  DelayLength=1  InitialCondition=0
  Gain1 : Gain  Gain=0.5000
  Subsystem : Subsystem
  Upsample2 : dspsigops/Upsample  N=2  phase=0  InputProcessing=Columns as channels (frame based)  RateOptions=Enforce single-rate processing  ic=0  mode=Unused parameter value
  Upsample3 : dspsigops/Upsample  N=2  phase=0  InputProcessing=Columns as channels (frame based)  RateOptions=Enforce single-rate processing  ic=0  mode=Unused parameter value
  Out1 : Outport
  wires:
  Upsample2/1 -> Delay4/1
  In1/1 -> Subsystem/1(In1), Delay3/1
  Gain1/1 -> Upsample2/1
  Add1/1 -> Out1/1
  Delay3/1 -> Gain1/1
  Upsample3/1 -> Add1/1
  Delay4/1 -> Add1/2
  Subsystem/1(Out1) -> Upsample3/1

== system fixed_point_model/Subsystem4/stage_5 ==
  In1 : Inport
  Add1 : Sum
  Delay3 : Delay  DelayLength=4  InitialCondition=0
  Delay4 : Delay  DelayLength=1  InitialCondition=0
  Gain1 : Gain  Gain=0.5000
  Subsystem : Subsystem
  Upsample2 : dspsigops/Upsample  N=2  phase=0  InputProcessing=Columns as channels (frame based)  RateOptions=Enforce single-rate processing  ic=0  mode=Unused parameter value
  Upsample3 : dspsigops/Upsample  N=2  phase=0  InputProcessing=Columns as channels (frame based)  RateOptions=Enforce single-rate processing  ic=0  mode=Unused parameter value
  Out1 : Outport
  wires:
  Upsample2/1 -> Delay4/1
  In1/1 -> Subsystem/1(In1), Delay3/1
  Gain1/1 -> Upsample2/1
  Add1/1 -> Out1/1
  Delay3/1 -> Gain1/1
  Upsample3/1 -> Add1/1
  Delay4/1 -> Add1/2
  Subsystem/1(Out1) -> Upsample3/1

== system fixed_point_model/Subsystem5/Sine Wave ==
  ReplicaOfSource : dspsrcs4/Sine Wave  Amplitude=0.631  Frequency=100e3  Phase=0  SampleMode=Discrete  OutComplex=Real  CompMethod=Trigonometric fcn  TableSize=Speed  SampleTime=1/3.125e6  SamplesPerFrame=1  ResetState=Restart at time zero  OutputFrames=off  dataType=double  wordLen=16  udDataType=sfix(16)  fracBitsMode=Best precision  numFracBits=15  OutDataTypeStr=double  LastOutDataTypeStr=double
  I : Outport  LockScale=on
  wires:
  ReplicaOfSource/1 -> I/1

== system fixed_point_model/Subsystem5/Sine Wave1 ==
  ReplicaOfSource : dspsrcs4/Sine Wave  Amplitude=0.631  Frequency=100e3  Phase=pi/2  SampleMode=Discrete  OutComplex=Real  CompMethod=Trigonometric fcn  TableSize=Speed  SampleTime=1/3.125e6  SamplesPerFrame=1  ResetState=Restart at time zero  OutputFrames=off  dataType=double  wordLen=16  udDataType=sfix(16)  fracBitsMode=Best precision  numFracBits=15  OutDataTypeStr=double  LastOutDataTypeStr=double
  Q : Outport  LockScale=on
  wires:
  ReplicaOfSource/1 -> Q/1

== system fixed_point_model/Subsystem5/Subsystem ==
  Q : Inport
  In2 : Inport  Port=2
  -I(t) : Gain  Gain=-1
  -Q(t) : Gain  Gain=-1
  Counter : simulink/Sources/Counter Limited  uplimit=3  tsamp=1/400e6
  Multiport Switch (MUX) : MultiPortSwitch  DataPortOrder=Zero-based contiguous  Inputs=4  zeroidx=on  SaturateOnIntegerOverflow=off  InputSameDT=off
  Out1 : Outport
  wires:
  Q/1 -> Multiport Switch (MUX)/2, -I(t)/1
  Counter/1 -> Multiport Switch (MUX)/1
  -Q(t)/1 -> Multiport Switch (MUX)/3
  In2/1 -> Multiport Switch (MUX)/5, -Q(t)/1
  -I(t)/1 -> Multiport Switch (MUX)/4
  Multiport Switch (MUX)/1 -> Out1/1

== system fixed_point_model/Subsystem5/Subsystem1 ==
  I : Inport
  Q : Inport  Port=2
  cos : Inport  Port=3
  sin : Inport  Port=4
  Add : Sum  Inputs=+-
  Product{,1..3} (4 alike) : Product
  Subtract : Sum
  Q' : Outport
  I' : Outport  Port=2
  wires:
  sin/1 -> Product/2, Product1/2
  Add/1 -> Q'/1
  Product3/1 -> Add/1
  Product2/1 -> Subtract/1
  Product1/1 -> Add/2
  Product/1 -> Subtract/2
  Subtract/1 -> I'/1
  I/1 -> Product1/1, Product2/2
  Q/1 -> Product3/2, Product/1
  cos/1 -> Product2/1, Product3/1

== system fixed_point_model/Subsystem5/Subsystem2 ==
  In1 : Inport
  Gain : Gain  Gain=2  SaturateOnIntegerOverflow=on
  Sign : Signum
  Sum : Sum  Inputs=|+-  RndMeth=Nearest  SaturateOnIntegerOverflow=on
  Sum1 : Sum  Inputs=|++-  SaturateOnIntegerOverflow=on
  Unit Delay : UnitDelay  InputProcessing=Columns as channels (frame based)  SampleTime=1e-8  HasFrameUpgradeWarning=on
  Unit Delay1 : UnitDelay  InputProcessing=Columns as channels (frame based)  SampleTime=1e-8  HasFrameUpgradeWarning=on
  Q : Outport
  wires:
  Sign/1 -> Q/1, Sum/2
  Sum1/1 -> Sign/1, Sum/1
  Sum/1 -> Unit Delay1/1
  Unit Delay1/1 -> Unit Delay/1, Gain/1
  Gain/1 -> Sum1/2
  In1/1 -> Sum1/1
  Unit Delay/1 -> Sum1/3

== system fixed_point_model/Subsystem5/Subsystem3 ==
  In1 : Inport
  Gain : Gain  Gain=2  SaturateOnIntegerOverflow=on
  Sign : Signum
  Sum : Sum  Inputs=|+-  RndMeth=Nearest  SaturateOnIntegerOverflow=on
  Sum1 : Sum  Inputs=|++-  SaturateOnIntegerOverflow=on
  Unit Delay : UnitDelay  InputProcessing=Columns as channels (frame based)  SampleTime=1e-8  HasFrameUpgradeWarning=on
  Unit Delay1 : UnitDelay  InputProcessing=Columns as channels (frame based)  SampleTime=1e-8  HasFrameUpgradeWarning=on
  Q : Outport
  wires:
  Sign/1 -> Q/1, Sum/2
  Sum1/1 -> Sign/1, Sum/1
  Sum/1 -> Unit Delay1/1
  Unit Delay1/1 -> Unit Delay/1, Gain/1
  Gain/1 -> Sum1/2
  In1/1 -> Sum1/1
  Unit Delay/1 -> Sum1/3

== system fixed_point_model/Subsystem5/filter_with_comb1 ==
  Q'1 : Inport
  Gain : Gain  Gain=1/512
  Stage_1 : Subsystem
  stage_3 : Subsystem
  stage_4 : Subsystem
  I' : Outport
  wires:
  stage_4/1(Out1) -> stage_3/1(In1)
  stage_3/1(Q') -> Stage_1/1(In1)
  Stage_1/1(Out1) -> Gain/1
  Gain/1 -> I'/1
  Q'1/1 -> stage_4/1(Q')

== system fixed_point_model/Subsystem5/filter_with_comb2 ==
  Q'1 : Inport
  Gain : Gain  Gain=1/512
  Stage_1 : Subsystem
  stage_3 : Subsystem
  stage_4 : Subsystem
  I' : Outport
  wires:
  stage_4/1(Out1) -> stage_3/1(In1)
  stage_3/1(Q') -> Stage_1/1(In1)
  Stage_1/1(Out1) -> Gain/1
  Gain/1 -> I'/1
  Q'1/1 -> stage_4/1(Q')

== system fixed_point_model/Subsystem6/Sine Wave ==
  ReplicaOfSource : dspsrcs4/Sine Wave  Amplitude=0.631  Frequency=100e3  Phase=0  SampleMode=Discrete  OutComplex=Real  CompMethod=Trigonometric fcn  TableSize=Speed  SampleTime=1/3.125e6  SamplesPerFrame=1  ResetState=Restart at time zero  OutputFrames=off  dataType=double  wordLen=16  udDataType=sfix(16)  fracBitsMode=Best precision  numFracBits=15  OutDataTypeStr=double  LastOutDataTypeStr=double
  I : Outport  LockScale=on
  wires:
  ReplicaOfSource/1 -> I/1

== system fixed_point_model/Subsystem6/Sine Wave1 ==
  ReplicaOfSource : dspsrcs4/Sine Wave  Amplitude=0.631  Frequency=100e3  Phase=pi/2  SampleMode=Discrete  OutComplex=Real  CompMethod=Trigonometric fcn  TableSize=Speed  SampleTime=1/3.125e6  SamplesPerFrame=1  ResetState=Restart at time zero  OutputFrames=off  dataType=double  wordLen=16  udDataType=sfix(16)  fracBitsMode=Best precision  numFracBits=15  OutDataTypeStr=double  LastOutDataTypeStr=double
  Q : Outport  LockScale=on
  wires:
  ReplicaOfSource/1 -> Q/1

== system fixed_point_model/Subsystem6/Subsystem ==
  Q : Inport
  In2 : Inport  Port=2
  -I(t) : Gain  Gain=-1
  -Q(t) : Gain  Gain=-1
  Counter : simulink/Sources/Counter Limited  uplimit=3  tsamp=1/400e6
  Multiport Switch (MUX) : MultiPortSwitch  DataPortOrder=Zero-based contiguous  Inputs=4  zeroidx=on  SaturateOnIntegerOverflow=off  InputSameDT=off
  Out1 : Outport
  wires:
  Q/1 -> Multiport Switch (MUX)/2, -I(t)/1
  Counter/1 -> Multiport Switch (MUX)/1
  -Q(t)/1 -> Multiport Switch (MUX)/3
  In2/1 -> Multiport Switch (MUX)/5, -Q(t)/1
  -I(t)/1 -> Multiport Switch (MUX)/4
  Multiport Switch (MUX)/1 -> Out1/1

== system fixed_point_model/Subsystem6/Subsystem1 ==
  I : Inport
  Q : Inport  Port=2
  cos : Inport  Port=3
  sin : Inport  Port=4
  Add : Sum  Inputs=+-
  Product{,1..3} (4 alike) : Product
  Subtract : Sum
  Q' : Outport
  I' : Outport  Port=2
  wires:
  sin/1 -> Product/2, Product1/2
  Add/1 -> Q'/1
  Product3/1 -> Add/1
  Product2/1 -> Subtract/1
  Product1/1 -> Add/2
  Product/1 -> Subtract/2
  Subtract/1 -> I'/1
  I/1 -> Product1/1, Product2/2
  Q/1 -> Product3/2, Product/1
  cos/1 -> Product2/1, Product3/1

== system fixed_point_model/Subsystem6/Subsystem2 ==
  In1 : Inport
  Gain : Gain  Gain=2  SaturateOnIntegerOverflow=on
  Sign : Signum
  Sum : Sum  Inputs=|+-  RndMeth=Nearest  SaturateOnIntegerOverflow=on
  Sum1 : Sum  Inputs=|++-  SaturateOnIntegerOverflow=on
  Unit Delay : UnitDelay  InputProcessing=Columns as channels (frame based)  SampleTime=1e-8  HasFrameUpgradeWarning=on
  Unit Delay1 : UnitDelay  InputProcessing=Columns as channels (frame based)  SampleTime=1e-8  HasFrameUpgradeWarning=on
  Q : Outport
  wires:
  Sign/1 -> Q/1, Sum/2
  Sum1/1 -> Sign/1, Sum/1
  Sum/1 -> Unit Delay1/1
  Unit Delay1/1 -> Unit Delay/1, Gain/1
  Gain/1 -> Sum1/2
  In1/1 -> Sum1/1
  Unit Delay/1 -> Sum1/3

== system fixed_point_model/Subsystem6/Subsystem3 ==
  In1 : Inport
  Gain : Gain  Gain=2  SaturateOnIntegerOverflow=on
  Sign : Signum
  Sum : Sum  Inputs=|+-  RndMeth=Nearest  SaturateOnIntegerOverflow=on
  Sum1 : Sum  Inputs=|++-  SaturateOnIntegerOverflow=on
  Unit Delay : UnitDelay  InputProcessing=Columns as channels (frame based)  SampleTime=1e-8  HasFrameUpgradeWarning=on
  Unit Delay1 : UnitDelay  InputProcessing=Columns as channels (frame based)  SampleTime=1e-8  HasFrameUpgradeWarning=on
  Q : Outport
  wires:
  Sign/1 -> Q/1, Sum/2
  Sum1/1 -> Sign/1, Sum/1
  Sum/1 -> Unit Delay1/1
  Unit Delay1/1 -> Unit Delay/1, Gain/1
  Gain/1 -> Sum1/2
  In1/1 -> Sum1/1
  Unit Delay/1 -> Sum1/3

== system fixed_point_model/Subsystem6/filter_with_comb1 ==
  Q'1 : Inport
  Gain : Gain  Gain=1/512
  Stage_1 : Subsystem
  stage_3 : Subsystem
  stage_4 : Subsystem
  I' : Outport
  wires:
  stage_4/1(Out1) -> stage_3/1(In1)
  stage_3/1(Q') -> Stage_1/1(In1)
  Stage_1/1(Out1) -> Gain/1
  Gain/1 -> I'/1
  Q'1/1 -> stage_4/1(Q')

== system fixed_point_model/Subsystem6/filter_with_comb2 ==
  Q'1 : Inport
  Gain : Gain  Gain=1/512
  Stage_1 : Subsystem
  stage_3 : Subsystem
  stage_4 : Subsystem
  I' : Outport
  wires:
  stage_4/1(Out1) -> stage_3/1(In1)
  stage_3/1(Q') -> Stage_1/1(In1)
  Stage_1/1(Out1) -> Gain/1
  Gain/1 -> I'/1
  Q'1/1 -> stage_4/1(Q')

== system fixed_point_model/Subsystem7/Sine Wave ==
  ReplicaOfSource : dspsrcs4/Sine Wave  Amplitude=0.631  Frequency=100e3  Phase=0  SampleMode=Discrete  OutComplex=Real  CompMethod=Trigonometric fcn  TableSize=Speed  SampleTime=1/3.125e6  SamplesPerFrame=1  ResetState=Restart at time zero  OutputFrames=off  dataType=double  wordLen=16  udDataType=sfix(16)  fracBitsMode=Best precision  numFracBits=15  OutDataTypeStr=double  LastOutDataTypeStr=double
  I : Outport  LockScale=on
  wires:
  ReplicaOfSource/1 -> I/1

== system fixed_point_model/Subsystem7/Sine Wave1 ==
  ReplicaOfSource : dspsrcs4/Sine Wave  Amplitude=0.631  Frequency=100e3  Phase=pi/2  SampleMode=Discrete  OutComplex=Real  CompMethod=Trigonometric fcn  TableSize=Speed  SampleTime=1/3.125e6  SamplesPerFrame=1  ResetState=Restart at time zero  OutputFrames=off  dataType=double  wordLen=16  udDataType=sfix(16)  fracBitsMode=Best precision  numFracBits=15  OutDataTypeStr=double  LastOutDataTypeStr=double
  Q : Outport  LockScale=on
  wires:
  ReplicaOfSource/1 -> Q/1

== system fixed_point_model/Subsystem7/Subsystem ==
  Q : Inport
  In2 : Inport  Port=2
  -I(t) : Gain  Gain=-1
  -Q(t) : Gain  Gain=-1
  Counter : simulink/Sources/Counter Limited  uplimit=3  tsamp=1/400e6
  Multiport Switch (MUX) : MultiPortSwitch  DataPortOrder=Zero-based contiguous  Inputs=4  zeroidx=on  SaturateOnIntegerOverflow=off  InputSameDT=off
  Out1 : Outport
  wires:
  Q/1 -> Multiport Switch (MUX)/2, -I(t)/1
  Counter/1 -> Multiport Switch (MUX)/1
  -Q(t)/1 -> Multiport Switch (MUX)/3
  In2/1 -> Multiport Switch (MUX)/5, -Q(t)/1
  -I(t)/1 -> Multiport Switch (MUX)/4
  Multiport Switch (MUX)/1 -> Out1/1

== system fixed_point_model/Subsystem7/Subsystem1 ==
  I : Inport
  Q : Inport  Port=2
  cos : Inport  Port=3
  sin : Inport  Port=4
  Add : Sum  Inputs=+-
  Product{,1..3} (4 alike) : Product
  Subtract : Sum
  Q' : Outport
  I' : Outport  Port=2
  wires:
  sin/1 -> Product/2, Product1/2
  Add/1 -> Q'/1
  Product3/1 -> Add/1
  Product2/1 -> Subtract/1
  Product1/1 -> Add/2
  Product/1 -> Subtract/2
  Subtract/1 -> I'/1
  I/1 -> Product1/1, Product2/2
  Q/1 -> Product3/2, Product/1
  cos/1 -> Product2/1, Product3/1

== system fixed_point_model/Subsystem7/Subsystem2 ==
  In1 : Inport
  Gain : Gain  Gain=2  SaturateOnIntegerOverflow=on
  Sign : Signum
  Sum : Sum  Inputs=|+-  RndMeth=Nearest  SaturateOnIntegerOverflow=on
  Sum1 : Sum  Inputs=|++-  SaturateOnIntegerOverflow=on
  Unit Delay : UnitDelay  InputProcessing=Columns as channels (frame based)  SampleTime=1e-8  HasFrameUpgradeWarning=on
  Unit Delay1 : UnitDelay  InputProcessing=Columns as channels (frame based)  SampleTime=1e-8  HasFrameUpgradeWarning=on
  Q : Outport
  wires:
  Sign/1 -> Q/1, Sum/2
  Sum1/1 -> Sign/1, Sum/1
  Sum/1 -> Unit Delay1/1
  Unit Delay1/1 -> Unit Delay/1, Gain/1
  Gain/1 -> Sum1/2
  In1/1 -> Sum1/1
  Unit Delay/1 -> Sum1/3

== system fixed_point_model/Subsystem7/Subsystem3 ==
  In1 : Inport
  Gain : Gain  Gain=2  SaturateOnIntegerOverflow=on
  Sign : Signum
  Sum : Sum  Inputs=|+-  RndMeth=Nearest  SaturateOnIntegerOverflow=on
  Sum1 : Sum  Inputs=|++-  SaturateOnIntegerOverflow=on
  Unit Delay : UnitDelay  InputProcessing=Columns as channels (frame based)  SampleTime=1e-8  HasFrameUpgradeWarning=on
  Unit Delay1 : UnitDelay  InputProcessing=Columns as channels (frame based)  SampleTime=1e-8  HasFrameUpgradeWarning=on
  Q : Outport
  wires:
  Sign/1 -> Q/1, Sum/2
  Sum1/1 -> Sign/1, Sum/1
  Sum/1 -> Unit Delay1/1
  Unit Delay1/1 -> Unit Delay/1, Gain/1
  Gain/1 -> Sum1/2
  In1/1 -> Sum1/1
  Unit Delay/1 -> Sum1/3

== system fixed_point_model/Subsystem7/filter_with_comb1 ==
  Q'1 : Inport
  Gain : Gain  Gain=1/512
  Stage_1 : Subsystem
  stage_3 : Subsystem
  stage_4 : Subsystem
  I' : Outport
  wires:
  stage_4/1(Out1) -> stage_3/1(In1)
  stage_3/1(Q') -> Stage_1/1(In1)
  Stage_1/1(Out1) -> Gain/1
  Gain/1 -> I'/1
  Q'1/1 -> stage_4/1(Q')

== system fixed_point_model/Subsystem7/filter_with_comb2 ==
  Q'1 : Inport
  Gain : Gain  Gain=1/512
  Stage_1 : Subsystem
  stage_3 : Subsystem
  stage_4 : Subsystem
  I' : Outport
  wires:
  stage_4/1(Out1) -> stage_3/1(In1)
  stage_3/1(Q') -> Stage_1/1(In1)
  Stage_1/1(Out1) -> Gain/1
  Gain/1 -> I'/1
  Q'1/1 -> stage_4/1(Q')

== system fixed_point_model/Subsystem8/Sine Wave ==
  ReplicaOfSource : dspsrcs4/Sine Wave  Amplitude=0.631  Frequency=100e3  Phase=0  SampleMode=Discrete  OutComplex=Real  CompMethod=Trigonometric fcn  TableSize=Speed  SampleTime=1/3.125e6  SamplesPerFrame=1  ResetState=Restart at time zero  OutputFrames=off  dataType=double  wordLen=16  udDataType=sfix(16)  fracBitsMode=Best precision  numFracBits=15  OutDataTypeStr=double  LastOutDataTypeStr=double
  I : Outport  LockScale=on
  wires:
  ReplicaOfSource/1 -> I/1

== system fixed_point_model/Subsystem8/Sine Wave1 ==
  ReplicaOfSource : dspsrcs4/Sine Wave  Amplitude=0.631  Frequency=100e3  Phase=pi/2  SampleMode=Discrete  OutComplex=Real  CompMethod=Trigonometric fcn  TableSize=Speed  SampleTime=1/3.125e6  SamplesPerFrame=1  ResetState=Restart at time zero  OutputFrames=off  dataType=double  wordLen=16  udDataType=sfix(16)  fracBitsMode=Best precision  numFracBits=15  OutDataTypeStr=double  LastOutDataTypeStr=double
  Q : Outport  LockScale=on
  wires:
  ReplicaOfSource/1 -> Q/1

== system fixed_point_model/Subsystem8/Subsystem ==
  Q : Inport
  In2 : Inport  Port=2
  -I(t) : Gain  Gain=-1
  -Q(t) : Gain  Gain=-1
  Counter : simulink/Sources/Counter Limited  uplimit=3  tsamp=1/400e6
  Multiport Switch (MUX) : MultiPortSwitch  DataPortOrder=Zero-based contiguous  Inputs=4  zeroidx=on  SaturateOnIntegerOverflow=off  InputSameDT=off
  Out1 : Outport
  wires:
  Q/1 -> Multiport Switch (MUX)/2, -I(t)/1
  Counter/1 -> Multiport Switch (MUX)/1
  -Q(t)/1 -> Multiport Switch (MUX)/3
  In2/1 -> Multiport Switch (MUX)/5, -Q(t)/1
  -I(t)/1 -> Multiport Switch (MUX)/4
  Multiport Switch (MUX)/1 -> Out1/1

== system fixed_point_model/Subsystem8/Subsystem1 ==
  I : Inport
  Q : Inport  Port=2
  cos : Inport  Port=3
  sin : Inport  Port=4
  Add : Sum  Inputs=+-
  Product{,1..3} (4 alike) : Product
  Subtract : Sum
  Q' : Outport
  I' : Outport  Port=2
  wires:
  sin/1 -> Product/2, Product1/2
  Add/1 -> Q'/1
  Product3/1 -> Add/1
  Product2/1 -> Subtract/1
  Product1/1 -> Add/2
  Product/1 -> Subtract/2
  Subtract/1 -> I'/1
  I/1 -> Product1/1, Product2/2
  Q/1 -> Product3/2, Product/1
  cos/1 -> Product2/1, Product3/1

== system fixed_point_model/Subsystem8/Subsystem2 ==
  In1 : Inport
  Gain : Gain  Gain=2  SaturateOnIntegerOverflow=on
  Sign : Signum
  Sum : Sum  Inputs=|+-  RndMeth=Nearest  SaturateOnIntegerOverflow=on
  Sum1 : Sum  Inputs=|++-  SaturateOnIntegerOverflow=on
  Unit Delay : UnitDelay  InputProcessing=Columns as channels (frame based)  SampleTime=1e-8  HasFrameUpgradeWarning=on
  Unit Delay1 : UnitDelay  InputProcessing=Columns as channels (frame based)  SampleTime=1e-8  HasFrameUpgradeWarning=on
  Q : Outport
  wires:
  Sign/1 -> Q/1, Sum/2
  Sum1/1 -> Sign/1, Sum/1
  Sum/1 -> Unit Delay1/1
  Unit Delay1/1 -> Unit Delay/1, Gain/1
  Gain/1 -> Sum1/2
  In1/1 -> Sum1/1
  Unit Delay/1 -> Sum1/3

== system fixed_point_model/Subsystem8/Subsystem3 ==
  In1 : Inport
  Gain : Gain  Gain=2  SaturateOnIntegerOverflow=on
  Sign : Signum
  Sum : Sum  Inputs=|+-  RndMeth=Nearest  SaturateOnIntegerOverflow=on
  Sum1 : Sum  Inputs=|++-  SaturateOnIntegerOverflow=on
  Unit Delay : UnitDelay  InputProcessing=Columns as channels (frame based)  SampleTime=1e-8  HasFrameUpgradeWarning=on
  Unit Delay1 : UnitDelay  InputProcessing=Columns as channels (frame based)  SampleTime=1e-8  HasFrameUpgradeWarning=on
  Q : Outport
  wires:
  Sign/1 -> Q/1, Sum/2
  Sum1/1 -> Sign/1, Sum/1
  Sum/1 -> Unit Delay1/1
  Unit Delay1/1 -> Unit Delay/1, Gain/1
  Gain/1 -> Sum1/2
  In1/1 -> Sum1/1
  Unit Delay/1 -> Sum1/3

== system fixed_point_model/Subsystem8/filter_with_comb1 ==
  Q'1 : Inport
  Gain : Gain  Gain=1/512
  Stage_1 : Subsystem
  stage_3 : Subsystem
  stage_4 : Subsystem
  I' : Outport
  wires:
  stage_4/1(Out1) -> stage_3/1(In1)
  stage_3/1(Q') -> Stage_1/1(In1)
  Stage_1/1(Out1) -> Gain/1
  Gain/1 -> I'/1
  Q'1/1 -> stage_4/1(Q')

== system fixed_point_model/Subsystem8/filter_with_comb2 ==
  Q'1 : Inport
  Gain : Gain  Gain=1/512
  Stage_1 : Subsystem
  stage_3 : Subsystem
  stage_4 : Subsystem
  I' : Outport
  wires:
  stage_4/1(Out1) -> stage_3/1(In1)
  stage_3/1(Q') -> Stage_1/1(In1)
  Stage_1/1(Out1) -> Gain/1
  Gain/1 -> I'/1
  Q'1/1 -> stage_4/1(Q')

== system fixed_point_model/Subsystem9/Sine Wave ==
  ReplicaOfSource : dspsrcs4/Sine Wave  Amplitude=0.631  Frequency=100e3  Phase=0  SampleMode=Discrete  OutComplex=Real  CompMethod=Trigonometric fcn  TableSize=Speed  SampleTime=1/3.125e6  SamplesPerFrame=1  ResetState=Restart at time zero  OutputFrames=off  dataType=double  wordLen=16  udDataType=sfix(16)  fracBitsMode=Best precision  numFracBits=15  OutDataTypeStr=double  LastOutDataTypeStr=double
  I : Outport  LockScale=on
  wires:
  ReplicaOfSource/1 -> I/1

== system fixed_point_model/Subsystem9/Sine Wave1 ==
  ReplicaOfSource : dspsrcs4/Sine Wave  Amplitude=0.631  Frequency=100e3  Phase=pi/2  SampleMode=Discrete  OutComplex=Real  CompMethod=Trigonometric fcn  TableSize=Speed  SampleTime=1/3.125e6  SamplesPerFrame=1  ResetState=Restart at time zero  OutputFrames=off  dataType=double  wordLen=16  udDataType=sfix(16)  fracBitsMode=Best precision  numFracBits=15  OutDataTypeStr=double  LastOutDataTypeStr=double
  Q : Outport  LockScale=on
  wires:
  ReplicaOfSource/1 -> Q/1

== system fixed_point_model/Subsystem9/Subsystem ==
  Q : Inport
  In2 : Inport  Port=2
  -I(t) : Gain  Gain=-1
  -Q(t) : Gain  Gain=-1
  Counter : simulink/Sources/Counter Limited  uplimit=3  tsamp=1/400e6
  Multiport Switch (MUX) : MultiPortSwitch  DataPortOrder=Zero-based contiguous  Inputs=4  zeroidx=on  SaturateOnIntegerOverflow=off  InputSameDT=off
  Out1 : Outport
  wires:
  Q/1 -> Multiport Switch (MUX)/2, -I(t)/1
  Counter/1 -> Multiport Switch (MUX)/1
  -Q(t)/1 -> Multiport Switch (MUX)/3
  In2/1 -> Multiport Switch (MUX)/5, -Q(t)/1
  -I(t)/1 -> Multiport Switch (MUX)/4
  Multiport Switch (MUX)/1 -> Out1/1

== system fixed_point_model/Subsystem9/Subsystem1 ==
  I : Inport
  Q : Inport  Port=2
  cos : Inport  Port=3
  sin : Inport  Port=4
  Add : Sum  Inputs=+-
  Product{,1..3} (4 alike) : Product
  Subtract : Sum
  Q' : Outport
  I' : Outport  Port=2
  wires:
  sin/1 -> Product/2, Product1/2
  Add/1 -> Q'/1
  Product3/1 -> Add/1
  Product2/1 -> Subtract/1
  Product1/1 -> Add/2
  Product/1 -> Subtract/2
  Subtract/1 -> I'/1
  I/1 -> Product1/1, Product2/2
  Q/1 -> Product3/2, Product/1
  cos/1 -> Product2/1, Product3/1

== system fixed_point_model/Subsystem9/Subsystem2 ==
  In1 : Inport
  Gain : Gain  Gain=2  SaturateOnIntegerOverflow=on
  Sign : Signum
  Sum : Sum  Inputs=|+-  RndMeth=Nearest  SaturateOnIntegerOverflow=on
  Sum1 : Sum  Inputs=|++-  SaturateOnIntegerOverflow=on
  Unit Delay : UnitDelay  InputProcessing=Columns as channels (frame based)  SampleTime=1e-8  HasFrameUpgradeWarning=on
  Unit Delay1 : UnitDelay  InputProcessing=Columns as channels (frame based)  SampleTime=1e-8  HasFrameUpgradeWarning=on
  Q : Outport
  wires:
  Sign/1 -> Q/1, Sum/2
  Sum1/1 -> Sign/1, Sum/1
  Sum/1 -> Unit Delay1/1
  Unit Delay1/1 -> Unit Delay/1, Gain/1
  Gain/1 -> Sum1/2
  In1/1 -> Sum1/1
  Unit Delay/1 -> Sum1/3

== system fixed_point_model/Subsystem9/Subsystem3 ==
  In1 : Inport
  Gain : Gain  Gain=2  SaturateOnIntegerOverflow=on
  Sign : Signum
  Sum : Sum  Inputs=|+-  RndMeth=Nearest  SaturateOnIntegerOverflow=on
  Sum1 : Sum  Inputs=|++-  SaturateOnIntegerOverflow=on
  Unit Delay : UnitDelay  InputProcessing=Columns as channels (frame based)  SampleTime=1e-8  HasFrameUpgradeWarning=on
  Unit Delay1 : UnitDelay  InputProcessing=Columns as channels (frame based)  SampleTime=1e-8  HasFrameUpgradeWarning=on
  Q : Outport
  wires:
  Sign/1 -> Q/1, Sum/2
  Sum1/1 -> Sign/1, Sum/1
  Sum/1 -> Unit Delay1/1
  Unit Delay1/1 -> Unit Delay/1, Gain/1
  Gain/1 -> Sum1/2
  In1/1 -> Sum1/1
  Unit Delay/1 -> Sum1/3

== system fixed_point_model/Subsystem9/filter_with_comb1 ==
  Q'1 : Inport
  Gain : Gain  Gain=1/512
  Stage_1 : Subsystem
  stage_3 : Subsystem
  stage_4 : Subsystem
  I' : Outport
  wires:
  stage_4/1(Out1) -> stage_3/1(In1)
  stage_3/1(Q') -> Stage_1/1(In1)
  Stage_1/1(Out1) -> Gain/1
  Gain/1 -> I'/1
  Q'1/1 -> stage_4/1(Q')

== system fixed_point_model/Subsystem9/filter_with_comb2 ==
  Q'1 : Inport
  Gain : Gain  Gain=1/512
  Stage_1 : Subsystem
  stage_3 : Subsystem
  stage_4 : Subsystem
  I' : Outport
  wires:
  stage_4/1(Out1) -> stage_3/1(In1)
  stage_3/1(Q') -> Stage_1/1(In1)
  Stage_1/1(Out1) -> Gain/1
  Gain/1 -> I'/1
  Q'1/1 -> stage_4/1(Q')
